simulink model "UrfcStorageSystem"  (R2026a)
settings: Solver=ode23t  StopTime=20040  MaxStep=5  RelTol=1e-4
model workspace (MAT data in the model file):
  urfcCurrentProfile = [0  0; 1200  0; 1260  300; 8460  300; 8520  0; 9120  0; 9180  -150; 19980  -150; 20040  0]
libraries: fl_lib x8, nesl_utility x6, greenH2_lib x2, slpidlib x1
settings Model: Creator=LENOVO  LastModifiedBy=LENOVO
settings SimscapeCC: SimscapeLogLimitData=off

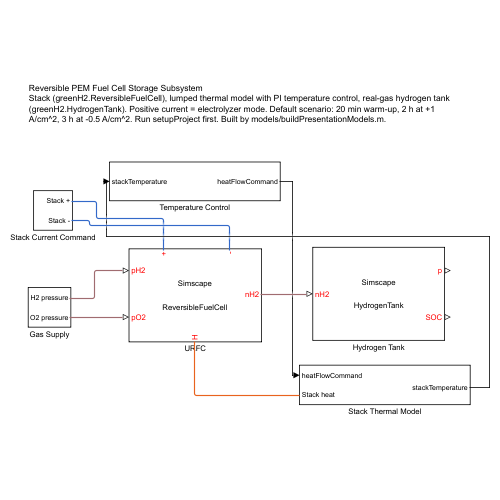
[thumbnail: Simulink's stored preview of the top-level diagram]
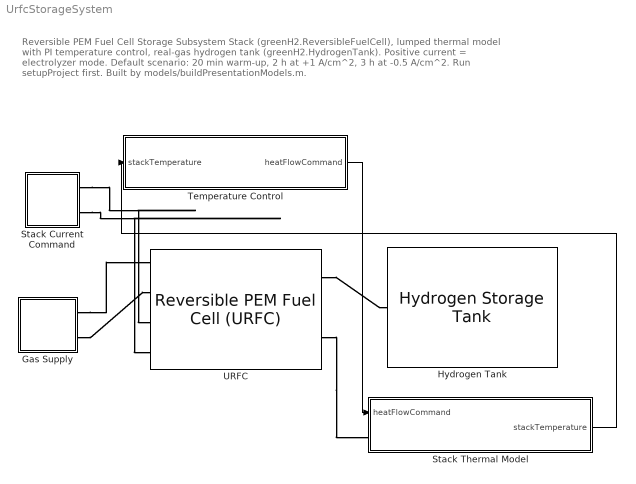
== system UrfcStorageSystem ==
  note: Reversible PEM Fuel Cell Storage Subsystem
      | Stack (greenH2.ReversibleFuelCell), lumped thermal model with PI temperature control, real-gas hydrogen tank
      | (greenH2.HydrogenTank). Positive current = electrolyzer mode. Default scenario: 20 min warm-up, 2 h at +1
      | A/cm^2, 3 h at -0.5 A/cm^2. Run setupProject first. Built by models/buildPresentationModels.m.
  Gas Supply : Subsystem
  Hydrogen Tank : greenH2_lib/Hydrogen Storage Tank  V_tank=0.5 m^3  T_tank=298.15 K  p_init=30 bar  p_min=5 bar  p_max=350 bar  b_H2=1.55e-05 m^3/mol  n_specify=off  n_priority=None  n=1000 mol  n_nominal_specify=off  n_nominal_value=1  n_nominal_unit=mol
  Stack Current Command : Subsystem
  Stack Thermal Model : Subsystem
  Temperature Control : Subsystem
  URFC : greenH2_lib/Reversible PEM Fuel Cell (URFC)  N_cell=100  A_cell=300 cm^2  t_mem=0.0050800000000000003 cm  lambda_EC=22  lambda_FC=10.109999999999999  R_contact=0.037440000000000001 Ohm*cm^2  j0_EC=0.0001009 A/cm^2  alpha_EC=0.5  j0_FC=1.4800000000000001e-05 A/cm^2  alpha_FC=0.5  gamma_O2=0.75149999999999995  E_a=0 J/mol  T_ref=353.14999999999998 K  jL_EC=20 A/cm^2  jL_FC=17.780000000000001 A/cm^2  psi_H2=8.2000000000000001e-11 mol/(cm*s*bar)  i_specify=off  i_priority=None  i=0 A  i_nominal_specify=off  i_nominal_value=1  i_nominal_unit=A  Q_specify=off  Q_priority=None  Q=0 W  Q_nominal_specify=off  Q_nominal_value=1  Q_nominal_unit=W
  wires:
  Temperature Control/1(heatFlowCommand) -> Stack Thermal Model/1(heatFlowCommand)
  Stack Thermal Model/1(stackTemperature) -> Temperature Control/1(stackTemperature)
  connections:
  Stack Current Command/RConn1 -- URFC/LConn3
  URFC/RConn2 -- Stack Thermal Model/LConn1
  Stack Current Command/RConn2 -- URFC/LConn4
  Gas Supply/RConn1 -- URFC/LConn1
  Gas Supply/RConn2 -- URFC/LConn2
  URFC/RConn1 -- Hydrogen Tank/LConn1

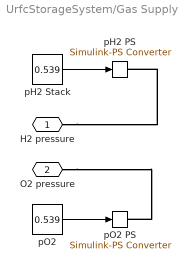
== system UrfcStorageSystem/Gas Supply ==
  pH2 PS : nesl_utility/Simulink-PS Converter  PhysicalDomain=network_engine_domain  SubClassName=ps_input  LeftPortType=input  RightPortType=output  PseudoPeriodic=off  Frequencies=[]  NoiseDistribution=none  NoiseParameters=[]  Unit=bar  AffineConversion=off  FilteringAndDerivatives=provide  SimscapeFilterOrder=1  InputFilterTimeConstant=0.001  UdotUserProvided=0
  pH2 Stack : Constant  Value=0.539
  pO2 : Constant  Value=0.539
  pO2 PS : nesl_utility/Simulink-PS Converter  PhysicalDomain=network_engine_domain  SubClassName=ps_input  LeftPortType=input  RightPortType=output  PseudoPeriodic=off  Frequencies=[]  NoiseDistribution=none  NoiseParameters=[]  Unit=bar  AffineConversion=off  FilteringAndDerivatives=provide  SimscapeFilterOrder=1  InputFilterTimeConstant=0.001  UdotUserProvided=0
  H2 pressure : PMIOPort  Side=Right
  O2 pressure : PMIOPort  Port=2  Side=Right
  wires:
  pH2 Stack/1 -> pH2 PS/1
  pO2/1 -> pO2 PS/1
  connections:
  O2 pressure/RConn1 -- pO2 PS/RConn1
  H2 pressure/RConn1 -- pH2 PS/RConn1

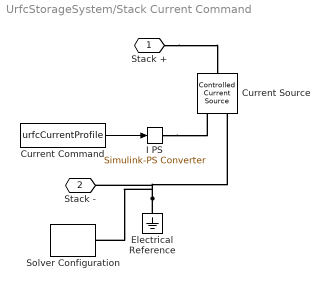
== system UrfcStorageSystem/Stack Current Command ==
  Current Command : FromWorkspace  VariableName=urfcCurrentProfile  OutputAfterFinalValue=Holding final value
  Current Source : fl_lib/Electrical/Electrical Sources/Controlled Current Source
  Electrical Reference : fl_lib/Electrical/Electrical Elements/Electrical Reference
  I PS : nesl_utility/Simulink-PS Converter  PhysicalDomain=network_engine_domain  SubClassName=ps_input  LeftPortType=input  RightPortType=output  PseudoPeriodic=off  Frequencies=[]  NoiseDistribution=none  NoiseParameters=[]  Unit=A  AffineConversion=off  FilteringAndDerivatives=provide  SimscapeFilterOrder=1  InputFilterTimeConstant=0.001  UdotUserProvided=0
  Solver Configuration : nesl_utility/Solver Configuration  PhysicalDomain=network_engine_domain  SubClassName=solver  LeftPortType=input  RightPortType=generic  Tones=[]  Harmonics=[]  SimulateNoise=off  Profile=off  UseLocalSampling=off  EnableSwitchedLinearOptims=on  FrequencyDomain=off  UseCCode=off  RelTol=0.001  AbsTol=0.001  MinStep=1e-09  ToWorkspace=off  RevertToSquareIcSolve=off  NumHomotopyIterations=100  PhasorMode=off  PhasorModeNumHarmonics=1  ConsistencySolver=NEWTON_XTOL_AFTER_FTOL  CanonicalOrdering=CANONICAL  OptimizeIntermediates=OPTIMIZED  IndexReductionMethod=DerivativeReplacement  DoDC=off  ResidualTolerance=1e-09  ConsistencyTolSource=GLOBAL  ConsistencyAbsTol=0.001  ConsistencyRelTol=0.001  ConsistencyTolFactor=0.001  UseLocalSolver=off  LocalSolverChoice=NE_BACKWARD_EULER_ADVANCER  ResolveIndetEquations=on  FunctionEvalNumThread=1  LocalSolverSampleTime=0.001  DoFixedCost=off  MaxNonlinIter=3  MaxModeIter=2  ComputeImpulses=off  ImpulseIterations=2  LinearAlgebra=auto  LinearAlgebraNumThread=0  EquationFormulation=NE_TIME_EF  DelaysMemoryBudget=1024  AutomaticFiltering=on  FilteringTimeConstant=0.001  PartitionStorageMethod=AS_NEEDED  PartitionMemoryBudget=1024  PartitionMethod=ROBUST  MultibodyUseLocalSolver=off  MultibodyLocalSolverChoice=ODE1  MultibodyLocalSolverSampleTime=0.001
  Stack + : PMIOPort  Side=Right
  Stack - : PMIOPort  Port=2  Side=Right
  wires:
  Current Command/1 -> I PS/1
  connections:
  Stack +/RConn1 -- Current Source/LConn1
  I PS/RConn1 -- Current Source/RConn1
  Electrical Reference/LConn1 -- Stack -/RConn1 -- Current Source/RConn2 -- Solver Configuration/RConn1

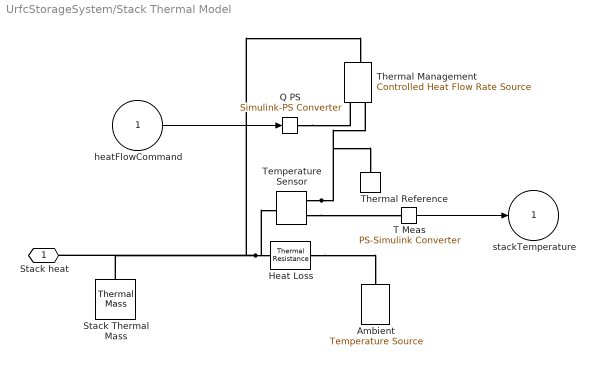
== system UrfcStorageSystem/Stack Thermal Model ==
  heatFlowCommand : Inport
  Ambient : fl_lib/Thermal/Thermal Sources/Temperature Source  temperature=298.15 K
  Heat Loss : fl_lib/Thermal/Thermal Elements/Thermal Resistance  resistance=0.06 K/W  T_specify=off  T_priority=None  T=0 K  T_nominal_specify=off  T_nominal_value=1  T_nominal_unit=K  Q_specify=off  Q_priority=None  Q=0 W  Q_nominal_specify=off  Q_nominal_value=1  Q_nominal_unit=W
  Q PS : nesl_utility/Simulink-PS Converter  PhysicalDomain=network_engine_domain  SubClassName=ps_input  LeftPortType=input  RightPortType=output  PseudoPeriodic=off  Frequencies=[]  NoiseDistribution=none  NoiseParameters=[]  Unit=W  AffineConversion=off  FilteringAndDerivatives=provide  SimscapeFilterOrder=1  InputFilterTimeConstant=0.001  UdotUserProvided=0
  Stack Thermal Mass : fl_lib/Thermal/Thermal Elements/Thermal Mass  mass_type=foundation.enum.constant_variable.constant  mass=57.69230769 kg  sp_heat=520 J/(kg*K)  mass_min=1e-6 kg  num_ports=foundation.enum.numPorts2.one  m_specify=off  m_priority=High  m=1 kg  m_nominal_specify=off  m_nominal_value=1  m_nominal_unit=kg  T_specify=on  T_priority=High  T=298.15 K  T_nominal_specify=off  T_nominal_value=1  T_nominal_unit=K  Q_specify=off  Q_priority=None  Q=0 W  Q_nominal_specify=off  Q_nominal_value=1  Q_nominal_unit=W
  T Meas : nesl_utility/PS-Simulink Converter  PhysicalDomain=network_engine_domain  SubClassName=ps_output  LeftPortType=input  RightPortType=output  PseudoPeriodic=off  Frequencies=[]  VectorFormat=inherit  Unit=K  AffineConversion=off
  Temperature Sensor : fl_lib/Thermal/Thermal Sensors/Temperature Sensor  temperature_measure=foundation.enum.MeasurementReference.difference
  Thermal Management : fl_lib/Thermal/Thermal Sources/Controlled Heat Flow Rate Source
  Thermal Reference : fl_lib/Thermal/Thermal Elements/Thermal Reference
  Stack heat : PMIOPort  Side=Left
  stackTemperature : Outport
  wires:
  heatFlowCommand/1 -> Q PS/1
  T Meas/1 -> stackTemperature/1
  connections:
  Stack Thermal Mass/LConn1 -- Stack heat/RConn1 -- Heat Loss/LConn1 -- Temperature Sensor/LConn1 -- Thermal Management/LConn1
  Q PS/RConn1 -- Thermal Management/RConn1
  Temperature Sensor/RConn1 -- Thermal Management/RConn2 -- Thermal Reference/LConn1
  Heat Loss/RConn1 -- Ambient/LConn1
  Temperature Sensor/RConn2 -- T Meas/LConn1

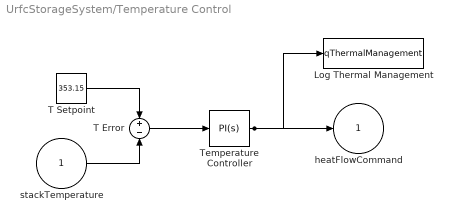
== system UrfcStorageSystem/Temperature Control ==
  stackTemperature : Inport
  Log Thermal Management : ToWorkspace  VariableName=qThermalManagement  SaveFormat=Timeseries  SampleTime=-1
  T Error : Sum  Inputs=+-
  T Setpoint : Constant  Value=353.15
  Temperature Controller : slpidlib/PID Controller  Controller=PI  Form=Parallel  TimeDomain=Continuous-time  UseExternalTs=off  SampleTime=-1  IntegratorMethod=Forward Euler  FilterMethod=Forward Euler  ControllerParametersSource=internal  P=3000  I=75  UseKiTs=off  D=0  UseExternalDerivativeSource=off  N=100  UseFilter=on  TunerSelectOption=Transfer Function Based (PID Tuner App)  InitialConditionSource=internal  InitialConditionForIntegrator=0  InitialConditionForFilter=0  DifferentiatorICPrevScaledInput=0  ExternalReset=none  TrackingMode=off  Kt=1  LimitOutput=on  SatLimitsSource=internal  UpperSaturationLimit=5000  LowerSaturationLimit=-40000  LinearizeAsGain=on  AntiWindupMode=clamping  Kb=1  LimitIntegrator=off  UpperIntegratorSaturationLimit=inf  LowerIntegratorSaturationLimit=-inf  POutMin=[]  POutMax=[]  IOutMin=[]  IOutMax=[]  DOutMin=[]  DOutMax=[]  NOutMin=[]  NOutMax=[]  SumOutMin=[]  SumOutMax=[]  SaturationOutMin=[]  SaturationOutMax=[]  PParamMin=[]  PParamMax=[]  IParamMin=[]  IParamMax=[]  DParamMin=[]  DParamMax=[]  NParamMin=[]  NParamMax=[]  KbParamMin=[]  KbParamMax=[]  KtParamMin=[]  KtParamMax=[]  KbOutMin=[]  KbOutMax=[]  KtOutMin=[]  KtOutMax=[]  IntegratorOutMin=[]  IntegratorOutMax=[]  FilterOutMin=[]  FilterOutMax=[]  SumI1OutMin=[]  SumI1OutMax=[]  SumI2OutMin=[]  SumI2OutMax=[]  SumI3OutMin=[]  SumI3OutMax=[]  SumI4OutMin=[]  SumI4OutMax=[]  SumDOutMin=[]  SumDOutMax=[]  DifferentiatorOutMin=[]  DifferentiatorOutMax=[]  FilterDiffOutCoefMin=[]  FilterDiffOutCoefMax=[]  ReciprocalOutMin=[]  ReciprocalOutMax=[]  SumDenOutMin=[]  SumDenOutMax=[]  SumNumOutMin=[]  SumNumOutMax=[]  DivideOutMin=[]  DivideOutMax=[]  UdiffTsProdOutMin=[]  UdiffTsProdOutMax=[]  NTsProdOutMin=[]  NTsProdOutMax=[]  UintegralTsProdOutMin=[]  UintegralTsProdOutMax=[]  UngainTsProdOutMin=[]  UngainTsProdOutMax=[]  ClampingZeroOutDataTypeStr=Inherit: Inherit via back propagation  ClampingZeroOutMin=[]  ClampingZeroOutMax=[]  FilterDenConstantOutDataTypeStr=Inherit: Inherit via back propagation  FilterDenConstantOutMin=[]  FilterDenConstantOutMax=[]  PCopyOutDataTypeStr=Inherit: Inherit via back propagation  PCopyOutMin=[]  PCopyOutMax=[]  NCopyOutDataTypeStr=Inherit: Inherit via back propagation  NCopyOutMin=[]  NCopyOutMax=[]  IntegratorContinuousStateAttributes=''  IntegratorStateMustResolveToSignalObject=off  IntegratorRTWStateStorageClass=Auto  FilterContinuousStateAttributes=''  FilterStateMustResolveToSignalObject=off  FilterRTWStateStorageClass=Auto  ParallelPVariant=InternalParameters  IdealPVariant=Disabled  IVariant=InternalParameters  DVariant=Disabled  IntegratorVariant=Continuous  SatVariant=Enabled  AWVariant=ContClampingParallel  PCopyVariant=Disabled  TRVariant=Disabled  FdbkBlocksVariant=Forward  IdealPFdbkVariant=Disabled  SatFdbkVariant=Disabled  DerivativeFilterVariant=Disabled  NVariant=Disabled  NCopyVariant=Disabled_SignalSpec  FilterICVariant=Disabled  IntegratorICVariant=InternalICs  ExternalResetVariant=Disabled  TRSumVariant=Passthrough  SumFdbkVariant=Disabled  SumVariant=Sum_PI  TsampFilterVariant=InternalTs  TsampNgainVariant=Passthrough  TsampIntegralVariant=Disabled_SignalSpec  ExternalSaturationOutDataTypeStr=Inherit: Same as second input  DerivativeSourceVariant=Disabled  PreIntVariant=InternalPreInt
  heatFlowCommand : Outport
  wires:
  T Error/1 -> Temperature Controller/1
  T Setpoint/1 -> T Error/1
  stackTemperature/1 -> T Error/2
  Temperature Controller/1 -> heatFlowCommand/1, Log Thermal Management/1
